simulink model "HW3"  (R2022b)
settings: Solver=VariableStepAuto  StartTime=0.0  StopTime=200  FixedStep=0.0001  RelTol=1e-3
libraries: simulink x1
settings Model: Creator=ali14  LastModifiedBy=ali14

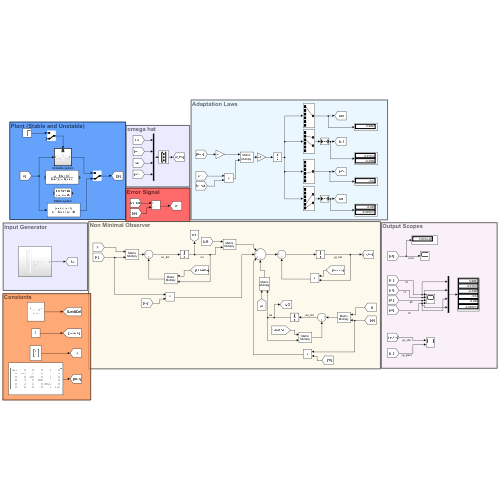
[thumbnail: Simulink's stored preview of the top-level diagram]
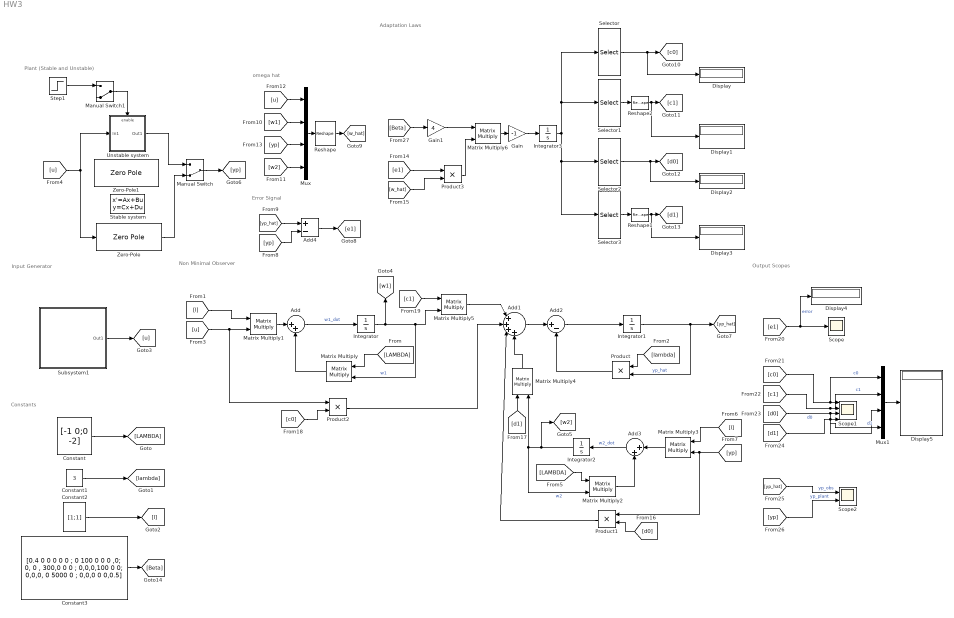
== system HW3 ==
  note: Plant (Stable and Unstable)
  note: Input Generator
  note: Constants
  note: Adaptation Laws
  note: Error Signal
  note: Non Minimal Observer
  note: omega hat
  note: Output Scopes
  Add : Sum  Inputs=|++
  Add1 : Sum  Inputs=|++++
  Add2 : Sum  Inputs=|+-
  Add3 : Sum  Inputs=|++
  Add4 : Sum  Inputs=+-
  Constant : Constant  Value=[-1 0;0 -2]  VectorParams1D=off
  Constant1 : Constant  Value=3
  Constant2 : Constant  Value=[1;1]  VectorParams1D=off
  Constant3 : Constant  Value="[0.4 0  0 0 0  0  ; 0  100  0 0 0 ,0;   0, 0 , 300,0 0 0   ;   0,0,0,100 0 0;   0,0,0, 0 5000 0  ;  0,0,0 0 0,0.5]"  VectorParams1D=off
  Display{,1..5} (6 alike) : Display
  Gain : Gain  Gain=-1
  Gain1 : Gain  Gain=4
  Integrator : Integrator  InitialCondition=[0;0]
  Integrator1 : Integrator
  Integrator2 : Integrator  InitialCondition=[0;0]
  Integrator3 : Integrator
  Manual Switch : ManualSwitch  CurrentSetting=0
  Manual Switch1 : ManualSwitch  CurrentSetting=0
  Matrix Multiply{,1..6} (7 alike) : Product  Multiplication=Matrix(*)
  Mux : Mux
  Mux1 : Mux
  Product{,1..3} (4 alike) : Product
  Reshape : Reshape  OutputDimensionality=Column vector (2-D)
  Reshape1 : Reshape  OutputDimensionality=Row vector (2-D)
  Reshape2 : Reshape  OutputDimensionality=Row vector (2-D)
  Scope : Scope
  Scope1 : Scope  NumInputPorts=4
  Scope2 : Scope  NumInputPorts=2
  Selector : Selector  InputPortWidth=6  IndexOptions=Index vector (dialog)  Indices=[1]  OutputSizes=1
  Selector1 : Selector  InputPortWidth=6  IndexOptions=Index vector (dialog)  Indices=[2 3]  OutputSizes=1
  Selector2 : Selector  InputPortWidth=6  IndexOptions=Index vector (dialog)  Indices=[4]  OutputSizes=1
  Selector3 : Selector  InputPortWidth=6  IndexOptions=Index vector (dialog)  Indices=[5 6]  OutputSizes=1
  Stable system : StateSpace  A=[0,0,-24;1 0 -26; 0 1 -9]  B=[1.5 ;2.5 ;1]  C=[0 0 1]  D=0  InitialCondition=[1 , 1.5,2]
  Step1 : Step  Time=0  SampleTime=0
  Subsystem1 : Subsystem
  Unstable system : Subsystem
  Zero-Pole : ZeroPole  Zeros=[-1,-1.5]  Poles="[-2  -3 -4]"  Gain=1
  Zero-Pole1 : ZeroPole  Zeros=[-1,-1.5]  Poles="[-2  3 -4]"  Gain=1
  wires:
  Mux1/1 -> Display5/1
  Subsystem1/1(Out1) -> [u]
  Gain1/1 -> Matrix Multiply6/1
  [Beta] -> Gain1/1
  Product3/1 -> Matrix Multiply6/2
  [w_hat] -> Product3/2
  [e1] -> Product3/1
  Constant3/1 -> [Beta]
  [yp] -> Scope2/2  "yp_plant"
  [yp_hat] -> Scope2/1  "yp_obs"
  Zero-Pole/1 -> Manual Switch/2
  [d1] -> Mux1/4, Scope1/4  "d1"
  [d0] -> Mux1/3, Scope1/3  "d0"
  [c1] -> Mux1/2, Scope1/2  "c1"
  [c0] -> Mux1/1, Scope1/1  "c0"
  [e1] -> Display4/1, Scope/1  "error"
  Step1/1 -> Manual Switch1/1
  Manual Switch1/1 -> Unstable system/Enable
  Unstable system/1(Out1) -> Manual Switch/1
  Manual Switch/1 -> [yp]
  Mux/1 -> Reshape/1
  Gain/1 -> Integrator3/1
  [LAMBDA] -> Matrix Multiply2/1
  Matrix Multiply/1 -> Add/2
  Selector3/1 -> Reshape1/1
  Selector2/1 -> Display2/1, [d0]
  Add2/1 -> Integrator1/1
  Reshape/1 -> [w_hat]
  [u] -> Zero-Pole/1, Unstable system/1(In1)
  Product/1 -> Add2/2
  [u] -> Mux/1
  [d1] -> Matrix Multiply4/1
  [c1] -> Matrix Multiply5/1
  Product2/1 -> Add1/2
  Add4/1 -> [e1]
  [yp_hat] -> Add4/1
  Selector1/1 -> Reshape2/1
  Product1/1 -> Add1/3
  Matrix Multiply5/1 -> Add1/1
  [c0] -> Product2/2
  [yp] -> Product1/1, Matrix Multiply3/2
  Integrator1/1 -> [yp_hat], Product/2  "yp_hat"
  Matrix Multiply1/1 -> Add/1
  [w1] -> Mux/2
  Reshape2/1 -> Display1/1, [c1]
  [u] -> Matrix Multiply1/2, Product2/1
  Constant1/1 -> [lambda]
  [l] -> Matrix Multiply1/1
  Matrix Multiply2/1 -> Add3/2
  Constant/1 -> [LAMBDA]
  Add1/1 -> Add2/1
  [yp] -> Add4/2
  Add/1 -> Integrator/1  "w1_dot"
  Matrix Multiply3/1 -> Add3/1
  [LAMBDA] -> Matrix Multiply/1
  Constant2/1 -> [l]
  Integrator3/1 -> Selector2/1, Selector3/1, Selector1/1, Selector/1
  Integrator2/1 -> [w2], Matrix Multiply2/2, Matrix Multiply4/2  "w2"
  Selector/1 -> Display/1, [c0]
  Add3/1 -> Integrator2/1  "w2_dot"
  [d0] -> Product1/2
  [l] -> Matrix Multiply3/1
  Matrix Multiply6/1 -> Gain/1
  [w2] -> Mux/4
  Matrix Multiply4/1 -> Add1/4
  [yp] -> Mux/3
  Reshape1/1 -> Display3/1, [d1]
  [lambda] -> Product/1
  Integrator/1 -> Matrix Multiply5/2, Matrix Multiply/2, [w1]  "w1"

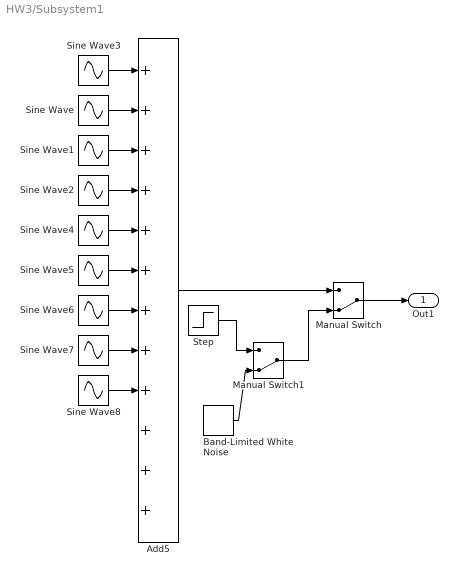
== system HW3/Subsystem1 ==
  Add5 : Sum  Inputs=++++++++++++
  Band-Limited White Noise : simulink/Sources/Band-Limited White Noise  Cov=[0.1]  Ts=0.1  seed=[23341]
  Manual Switch : ManualSwitch  CurrentSetting=0
  Manual Switch1 : ManualSwitch  CurrentSetting=0
  Sine Wave : Sin  Amplitude=7  SampleTime=0
  Sine Wave1 : Sin  Amplitude=5  Frequency=2  SampleTime=0
  Sine Wave2 : Sin  Frequency=3  SampleTime=0
  Sine Wave3 : Sin  Amplitude=10  Frequency=200  SampleTime=0
  Sine Wave4 : Sin  Amplitude=2  Frequency=17  SampleTime=0
  Sine Wave5 : Sin  Amplitude=5  Frequency=12  SampleTime=0
  Sine Wave6 : Sin  Amplitude=6  Frequency=44  SampleTime=0
  Sine Wave7 : Sin  Amplitude=5  Frequency=65  SampleTime=0
  Sine Wave8 : Sin  Amplitude=3  Frequency=0.1  SampleTime=0
  Step : Step  Time=0  SampleTime=0
  Out1 : Outport
  wires:
  Sine Wave2/1 -> Add5/4
  Sine Wave/1 -> Add5/2
  Sine Wave5/1 -> Add5/6
  Sine Wave1/1 -> Add5/3
  Sine Wave4/1 -> Add5/5
  Sine Wave3/1 -> Add5/1
  Sine Wave8/1 -> Add5/9
  Sine Wave7/1 -> Add5/8
  Sine Wave6/1 -> Add5/7
  Manual Switch/1 -> Out1/1
  Add5/1 -> Manual Switch/1
  Band-Limited White Noise/1 -> Manual Switch1/2
  Manual Switch1/1 -> Manual Switch/2
  Step/1 -> Manual Switch1/1

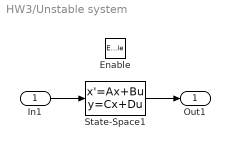
== system HW3/Unstable system ==
  In1 : Inport
  Enable : EnablePort
  State-Space1 : StateSpace  A=[0,0,24;1 0 10; 0 1 -3]  B=[1.5 ;2.5 ;1]  C=[0 0 1]  D=0  InitialCondition=[1 , 1.5,2]
  Out1 : Outport
  wires:
  In1/1 -> State-Space1/1
  State-Space1/1 -> Out1/1
